simulink model "es_4_model"  (R2024b)
settings: Solver=VariableStepAuto  StartTime=0.0  StopTime=20  RelTol=1e-3
values from neighbouring files (symbols this model uses):
  q_i = [alpha+1  1  pi/4]'    [es_4_main.m]
  Ts = 0.001    [es_4_main.m]
libraries: robotmobilelib x1
settings Model: Creator=feder  LastModifiedBy=feder

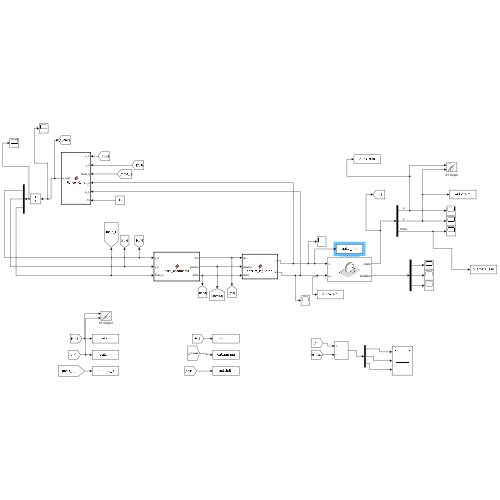
[thumbnail: Simulink's stored preview of the top-level diagram]
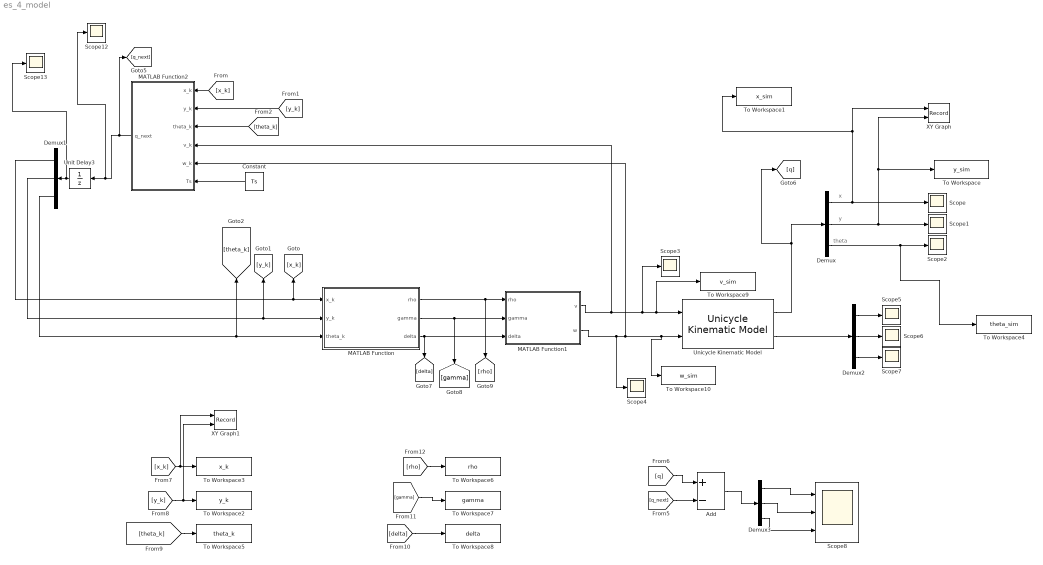
== system es_4_model ==
  note: theta
  note: y
  note: x
  Add : Sum  Inputs=+-
  Constant : Constant  Value=Ts
  Demux{,1..3} (4 alike) : Demux  Outputs=3
  MATLAB Function : MATLAB Function  TreatAsAtomicUnit=on
  MATLAB Function1 : MATLAB Function  TreatAsAtomicUnit=on
  MATLAB Function2 : MATLAB Function  TreatAsAtomicUnit=on
  Scope{,1..7,12..13} (10 alike) : Scope
  Scope8 : Scope  NumInputPorts=3
  To Workspace : ToWorkspace  VariableName=y_sim  SaveFormat=Timeseries  SampleTime=-1
  To Workspace1 : ToWorkspace  VariableName=x_sim  SaveFormat=Timeseries  SampleTime=-1
  To Workspace10 : ToWorkspace  VariableName=w_sim  SaveFormat=Timeseries  SampleTime=-1
  To Workspace2 : ToWorkspace  VariableName=y_k  SaveFormat=Timeseries  SampleTime=-1
  To Workspace3 : ToWorkspace  VariableName=x_k  SaveFormat=Timeseries  SampleTime=-1
  To Workspace4 : ToWorkspace  VariableName=theta_sim  SaveFormat=Timeseries  SampleTime=-1
  To Workspace5 : ToWorkspace  VariableName=theta_k  SaveFormat=Timeseries  SampleTime=-1
  To Workspace6 : ToWorkspace  VariableName=rho  SaveFormat=Timeseries  SampleTime=-1
  To Workspace7 : ToWorkspace  VariableName=gamma  SaveFormat=Timeseries  SampleTime=-1
  To Workspace8 : ToWorkspace  VariableName=delta  SaveFormat=Timeseries  SampleTime=-1
  To Workspace9 : ToWorkspace  VariableName=v_sim  SaveFormat=Timeseries  SampleTime=-1
  Unicycle Kinematic Model : robotmobilelib/Unicycle Kinematic Model  VehicleInputs=Vehicle Speed & Heading Angular Velocity  WheelRadius=0.1  WheelSpeedRange=[-Inf Inf]  InitialState=q_i  SimulateUsing=Interpreted execution
  Unit Delay3 : UnitDelay  InitialCondition=q_i  SampleTime=Ts  HasFrameUpgradeWarning=on
  XY Graph : Record  FileSettingsInternal="{\"entries\":[{\"content\":{\"excelSettings\":{\"content\":{},\"type\":\"Streamout.ExcelSettings\"}},\"type\":\"Streamout.FileSettingStorage\",\"uuid\":\"\"}],\"packageUris\":[\"http:\\/\\/schema.mathworks.com\\/mf0\\/streamout_blocks\\/R2020a\"],\"version\":\"1.0\"}"  Layout=[1 1]  SignalsInternal="{\"entries\":[{\"content\":{\"signals\":[{\"content\":{\"blockPath\":[],\"dimensions\":[1],\"domain\":\"\",\"lineColor\":\"#a2142f\",\"plots\":[ 1 ],\"port\":1,\"sid\":[\"\"],\"signalID\":1,\"signalName\":\"Demux:1\"},\"type\":\"RecordBlkView.Signal\",\"uuid\":\"\"},{\"content\":{\"blockPath\":[],\"dimensions\":[1],\"domain\":\"\",\"lineColor\":\"#139fff\",\"plots\":[ 1 ],\"port\":2,\"sid\":[\"\"],\"signalID\":2,\"signalName\":\"Demux:2\"},\"type\":\"RecordBlkView.Signal\",\"uuid\":\"\"}]},\"type\":\"RecordBlkView.InputSignals\",\"uuid\":\"\"}],\"packageUris\":[\"http:\\/\\/schema.mathworks.com\\/mf0\\/streamout_blocks\\/R2020a\"],\"version\":\"1.0\"}"  VisualizationBindings="{\"xyplotplugin\":{\"info\":[{\"series\":[{\"bindingParametersList\":[{\"parameter\":\"X-Axis\",\"signalID\":1,\"signalName\":\"Demux:1\"},{\"parameter\":\"Y-Axis\",\"signalID\":2,\"signalName\":\"Demux:2\"}],\"seriesID\":0}],\"subplotID\":1}]}}"  CompatibilityTag=XY
  XY Graph1 : Record  FileSettingsInternal="{\"entries\":[{\"content\":{\"excelSettings\":{\"content\":{},\"type\":\"Streamout.ExcelSettings\"}},\"type\":\"Streamout.FileSettingStorage\",\"uuid\":\"\"}],\"packageUris\":[\"http:\\/\\/schema.mathworks.com\\/mf0\\/streamout_blocks\\/R2020a\"],\"version\":\"1.0\"}"  Layout=[1 1]  SignalsInternal="{\"entries\":[{\"content\":{\"signals\":[{\"content\":{\"blockPath\":[],\"dimensions\":[1,1],\"domain\":\"\",\"lineColor\":\"#a2142f\",\"plots\":[ 1 ],\"port\":1,\"sid\":[\"\"],\"signalID\":1,\"signalName\":\"From7\"},\"type\":\"RecordBlkView.Signal\",\"uuid\":\"\"},{\"content\":{\"blockPath\":[],\"dimensions\":[1,1],\"domain\":\"\",\"lineColor\":\"#139fff\",\"plots\":[ 1 ],\"port\":2,\"sid\":[\"\"],\"signalID\":2,\"signalName\":\"From8\"},\"type\":\"RecordBlkView.Signal\",\"uuid\":\"\"}]},\"type\":\"RecordBlkView.InputSignals\",\"uuid\":\"\"}],\"packageUris\":[\"http:\\/\\/schema.mathworks.com\\/mf0\\/streamout_blocks\\/R2020a\"],\"version\":\"1.0\"}"  VisualizationBindings="{\"xyplotplugin\":{\"info\":[{\"series\":[{\"bindingParametersList\":[{\"parameter\":\"X-Axis\",\"signalID\":1,\"signalName\":\"From7\"},{\"parameter\":\"Y-Axis\",\"signalID\":2,\"signalName\":\"From8\"}],\"seriesID\":0}],\"subplotID\":1}]}}"  CompatibilityTag=XY
  wires:
  MATLAB Function/1(rho) -> [rho], MATLAB Function1/1(rho)
  MATLAB Function/2(gamma) -> MATLAB Function1/2(gamma), [gamma]
  MATLAB Function/3(delta) -> [delta], MATLAB Function1/3(delta)
  Constant/1 -> MATLAB Function2/6(Ts)
  MATLAB Function1/1(v) -> MATLAB Function2/4(v_k), Scope3/1, To Workspace9/1, Unicycle Kinematic Model/1
  MATLAB Function1/2(w) -> Scope4/1, MATLAB Function2/5(w_k), To Workspace10/1, Unicycle Kinematic Model/2
  Unicycle Kinematic Model/1 -> [q], Demux/1
  Demux/3 -> To Workspace4/1, Scope2/1
  Demux/2 -> XY Graph/2, To Workspace/1, Scope1/1
  Demux/1 -> To Workspace1/1, XY Graph/1, Scope/1
  Demux1/1 -> MATLAB Function/1(x_k), [x_k]
  Demux1/2 -> [y_k], MATLAB Function/2(y_k)
  Demux1/3 -> [theta_k], MATLAB Function/3(theta_k)
  [x_k] -> MATLAB Function2/1(x_k)
  Unit Delay3/1 -> Scope13/1, Demux1/1
  MATLAB Function2/1(q_next) -> [q_next], Unit Delay3/1, Scope12/1
  [y_k] -> MATLAB Function2/2(y_k)
  [theta_k] -> MATLAB Function2/3(theta_k)
  Unicycle Kinematic Model/2 -> Demux2/1
  Demux2/1 -> Scope5/1
  Demux2/2 -> Scope6/1
  Demux2/3 -> Scope7/1
  [q_next] -> Add/2
  [q] -> Add/1
  Add/1 -> Demux3/1
  Demux3/1 -> Scope8/1
  Demux3/2 -> Scope8/2
  Demux3/3 -> Scope8/3
  [x_k] -> XY Graph1/1, To Workspace3/1
  [y_k] -> XY Graph1/2, To Workspace2/1
  [theta_k] -> To Workspace5/1
  [gamma] -> To Workspace7/1
  [delta] -> To Workspace8/1
  [rho] -> To Workspace6/1

== matlab function es_4_model/MATLAB Function1 ==
  data: rho input; v output; gamma input; delta input; w output
function [v, w] = posture_regulation(rho, gamma, delta)

    k1=1;
    k2=50;
    k3=10;

     v = k1*rho*cos(gamma);
     w = k2*gamma + k1*sin(gamma)*cos(gamma)*(1+k3*delta/gamma);
end

== matlab function es_4_model/MATLAB Function ==
  data: x_k input; rho output; y_k input; theta_k input; gamma output; delta output
function [rho, gamma, delta] = polar_coordinates(x_k, y_k, theta_k)
    rho = sqrt(x_k^2 + y_k^2);
    gamma =  atan2(y_k, x_k) -theta_k +pi;
    delta = theta_k + gamma;
end

== matlab function es_4_model/MATLAB Function2 ==
  data: x_k input; y_k input; theta_k input; v_k input; w_k input; q_next output; Ts input
function q_next = Runge_Kutta(x_k, y_k, theta_k, v_k, w_k, Ts)
    % x = q(1);
    % y = q(2);
    % theta = q(3);

    theta_mid = theta_k + 0.5 * w_k * Ts;

    x_next = x_k + v_k * Ts * cos(theta_mid);
    y_next = y_k + v_k * Ts * sin(theta_mid);
    theta_next = theta_k + w_k * Ts;

    q_next = [x_next; y_next; theta_next];
end
